simulink model "P170_PV_MPPT_Integration"  (R2026b)
settings: Solver=FixedStepDiscrete  StopTime=2  FixedStep=P170_dt
values from neighbouring files (symbols this model uses):
  P170_Imp = im(ix)    [P170_PV_Initialize.m]
  P170_Vmp = vm(ix)    [P170_PV_Initialize.m]
undefined symbols (not defined in the file or in its folder): P170_T
libraries: fl_lib x4, nesl_utility x2, ee_lib x1
settings Model: Creator=simay  LastModifiedBy=aj26g
settings SimscapeCC: SimscapeLogType=all  SimscapeNominalValues="[{\"value\":\"1\",\"unit\":\"A\"},{\"value\":\"1\",\"unit\":\"bar\"},{\"value\":\"1\",\"unit\":\"cm^2\"},{\"value\":\"1\",\"unit\":\"cm^3/s\"},{\"value\":\"1\",\"unit\":\"kJ/kg\"},{\"value\":\"1\",\"unit\":\"kW\"},{\"value\":\"1\",\"unit\":\"l\"},{\"value\":\"1\",\"unit\":\"N\"},{\"value\":\"1\",\"unit\":\"N*m\"},{\"value\":\"1\",\"unit\":\"V\"},{\"value\":\"0.001\",\"unit\":\"Wb\"}]"  SimscapeUseEnergyAccounting=off

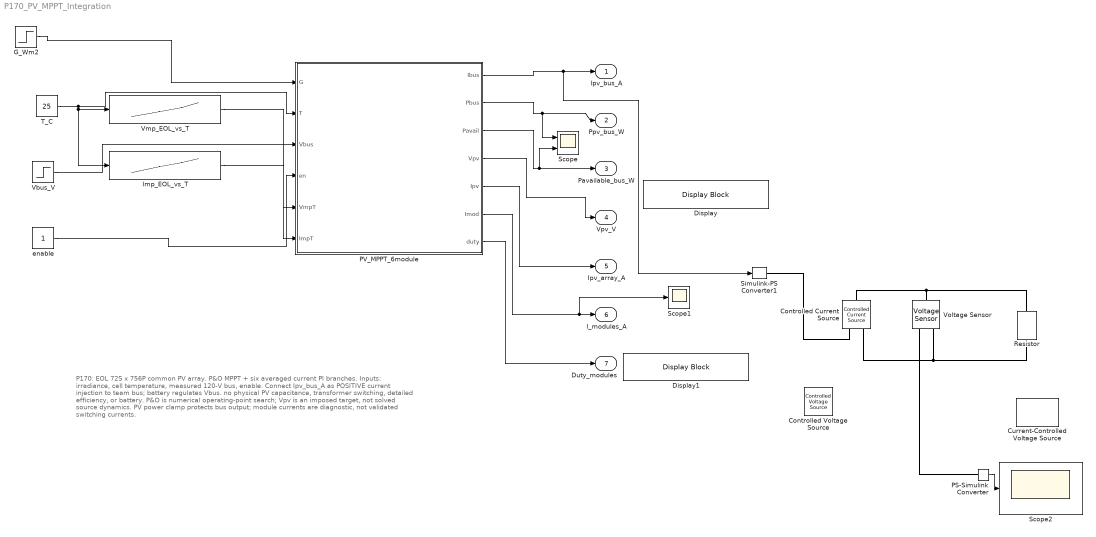
== system P170_PV_MPPT_Integration ==
  note: P170: EOL 72S x 756P common PV array. P&O MPPT + six averaged current PI branches.
      | Inputs: irradiance, cell temperature, measured 120-V bus, enable.
      | Connect Ipv_bus_A as POSITIVE current injection to team bus; battery regulates Vbus.
      |
      | no physical PV capacitance, transformer switching, detailed efficiency, or battery.
      | P&O is numerical operating-point search; Vpv is an imposed target, not solved source dynamics.
      | PV power clamp protects bus output; module currents are diagnostic, not validated switching currents.
  Controlled Current Source : fl_lib/Electrical/Electrical Sources/Controlled Current Source
  Controlled Voltage Source : fl_lib/Electrical/Electrical Sources/Controlled Voltage Source
  Current-Controlled Voltage Source : fl_lib/Electrical/Electrical Sources/Current-Controlled Voltage Source  K=1 Ohm  i1_specify=off  i1_priority=None  i1=0 A  i1_nominal_specify=off  i1_nominal_value=1  i1_nominal_unit=A  v2_specify=off  v2_priority=None  v2=0 V  v2_nominal_specify=off  v2_nominal_value=1  v2_nominal_unit=V
  Display : DisplayBlock  LabelPosition=Hide  Transparency=1  GridColor=[0.502, 0.502, 0.502]
  Display1 : DisplayBlock  LabelPosition=Hide  Transparency=1  GridColor=[0.502, 0.502, 0.502]
  G_Wm2 : Step  Time=0.8  InitialValue=1367  FinalValue=700  SampleTime=0
  Imp_EOL_vs_T : Lookup_n-D  NumberOfTableDimensions=1  BreakpointsForDimension1=P170_T  Table=P170_Imp  InternalRulePriority=Speed  RndMeth=Simplest
  PS-Simulink Converter : nesl_utility/PS-Simulink Converter  PhysicalDomain=network_engine_domain  SubClassName=ps_output  LeftPortType=input  RightPortType=output  PseudoPeriodic=off  Frequencies=[]  VectorFormat=inherit  Unit=inherit  AffineConversion=off
  PV_MPPT_6module : MATLAB Function  TreatAsAtomicUnit=on
  Resistor : ee_lib/Passive/Resistor  R=30000 Ohm  enable_R_tol=ee.enum.toleranceApplication.none  R_tol=5  tol_distribution=ee.enum.toleranceDistribution.uniform  nSigma=4  enable_operating_limits=ee.enum.enable.no  operating_limit_action=ee.enum.passive.reportOpLim.warn  power_rating=1 W  max_working_voltage=100 V  noise_mode=ee.enum.sources.noise.Disabled  Tdevice=25 degC  sample_time=1e-3 s  repeatability=ee.enum.ic.repeatability.notRepeatable  user_seed=0  auto_seed=4111000739  power_derating_T1=70 degC  power_derating_T2=155 degC  operating_temperature_range_vec=[-50, 150] degC  alpha=3.93e-3 1/K  Tmeas=25 degC  thermal_mass=100 J/K  temperature_specify=off  temperature_priority=High  temperature=298.15 K  temperature_nominal_specify=off  temperature_nominal_value=1  temperature_nominal_unit=K
  Scope : Scope  NumInputPorts=2
      settings: ActiveDisplayYMinimum=-1.4996053799360058  ActiveDisplayYMaximum=1.4239551585454688
  Scope1 : Scope
      settings: ActiveDisplayYMinimum=25.569170414602688  ActiveDisplayYMaximum=92.411823172385326
  Scope2 : Scope
      settings: DataLoggingVariableName=ScopeData2
  Simulink-PS Converter1 : nesl_utility/Simulink-PS Converter  PhysicalDomain=network_engine_domain  SubClassName=ps_input  LeftPortType=input  RightPortType=output  PseudoPeriodic=off  Frequencies=[]  NoiseDistribution=none  NoiseParameters=[]  Unit=1  AffineConversion=off  FilteringAndDerivatives=provide  SimscapeFilterOrder=1  InputFilterTimeConstant=0.001  UdotUserProvided=0
  T_C : Constant  Value=25
  Vbus_V : Step  Time=1.2  InitialValue=120  FinalValue=115  SampleTime=0
  Vmp_EOL_vs_T : Lookup_n-D  NumberOfTableDimensions=1  BreakpointsForDimension1=P170_T  Table=P170_Vmp  InternalRulePriority=Speed  RndMeth=Simplest
  Voltage Sensor : fl_lib/Electrical/Electrical Sensors/Voltage Sensor
  enable : Constant
  Ipv_bus_A : Outport
  Ppv_bus_W : Outport  Port=2
  Pavailable_bus_W : Outport  Port=3
  Vpv_V : Outport  Port=4
  Ipv_array_A : Outport  Port=5
  I_modules_A : Outport  Port=6
  Duty_modules : Outport  Port=7
  wires:
  G_Wm2/1 -> PV_MPPT_6module/1(G)
  T_C/1 -> Vmp_EOL_vs_T/1, Imp_EOL_vs_T/1, PV_MPPT_6module/2(T)
  Vbus_V/1 -> PV_MPPT_6module/3(Vbus)
  enable/1 -> PV_MPPT_6module/4(en)
  Vmp_EOL_vs_T/1 -> PV_MPPT_6module/5(VmpT)
  Imp_EOL_vs_T/1 -> PV_MPPT_6module/6(ImpT)
  PV_MPPT_6module/1(Ibus) -> Simulink-PS Converter1/1, Ipv_bus_A/1
  PV_MPPT_6module/3(Pavail) -> Scope/2, Pavailable_bus_W/1
  PV_MPPT_6module/4(Vpv) -> Vpv_V/1
  PV_MPPT_6module/5(Ipv) -> Ipv_array_A/1
  PV_MPPT_6module/6(Imod) -> Scope1/1, I_modules_A/1
  PV_MPPT_6module/7(duty) -> Duty_modules/1
  PV_MPPT_6module/2(Pbus) -> Scope/1, Ppv_bus_W/1
  PS-Simulink Converter/1 -> Scope2/1
  connections:
  Controlled Current Source/RConn1 -- Simulink-PS Converter1/RConn1
  Resistor/LConn1 -- Controlled Current Source/LConn1 -- Voltage Sensor/LConn1
  Controlled Current Source/RConn2 -- Voltage Sensor/RConn2 -- Resistor/RConn1
  PS-Simulink Converter/LConn1 -- Voltage Sensor/RConn1

== matlab function P170_PV_MPPT_Integration/PV_MPPT_6module ==
  data: G input; Ibus output; T input; Vbus input; en input; VmpT input; ImpT input; Pbus output; Pavail output; Vpv output; Ipv output; Imod output; duty output
function [Ibus, Pbus, Pavail, Vpv, Ipv, Imod, duty] = fcn(G,T,Vbus,en,VmpT,ImpT)
%#codegen
% EOL teammate MPP data; illustrative piecewise I-V fit.
% Shared PV bus, single coordinated P&O, six averaged PI branches.
persistent Vcmd dir Pprev count il integ
if isempty(Vcmd)
 Vcmd=217; dir=1; Pprev=0; count=0; il=zeros(6,1); integ=zeros(6,1);
end
dt=1e-4; eta=0.96; Gref=1367;
gs=max(0,min(1.5,G/Gref));
vmp=max(10,VmpT); imp=max(0,ImpT)*gs;
% Curve passes through Isc, Imp at Vmp, and zero at Voc.
% Isc=1.04 Imp, Voc=1.13 Vmp are MODEL ASSUMPTIONS.
isc=1.04*imp; voc=1.13*vmp;
Vcmd=max(0.5*vmp,min(0.99*voc,Vcmd));
if Vcmd<=vmp
 ipv=max(0,isc-(isc-imp)*(Vcmd/vmp)^2);
else
 ipv=max(0,imp*(voc-Vcmd)/(voc-vmp));
end
Ppv=Vcmd*ipv; Pavail=max(0,vmp*imp*eta);
count=count+1;
if count>=100
 if Ppv<Pprev, dir=-dir; end
 Vcmd=Vcmd+dir*0.5; Pprev=Ppv; count=0;
end
% Power-to-current reference; current limited by PV production.
v=max(30,Vbus);
Ptarget=max(0,min(Ppv*eta,Pavail))*max(0,min(1,en));
Iref=Ptarget/v/6;
Imod=zeros(6,1); duty=zeros(6,1);
for k=1:6
 % Averaged current PI with feedforward; shared-array duty proxy.
 err=Iref-il(k);
 dff=Vbus/max(1,1.15*Vcmd);
 d=max(0,min(0.85,dff+0.0015*err+integ(k)));
 % Average inductor dynamics; 33 uH each.
 next=il(k)+dt*(1.15*Vcmd*d-Vbus)/33e-6;
 % Avoid nonphysical reverse PV current.
 next=max(0,next);
 % Anti-windup: integrate only when unsaturated or correcting.
 if (d>0 && d<0.85) || (d<=0 && err>0) || (d>=0.85 && err<0)
  integ(k)=integ(k)+3*dt*err;
 end
 il(k)=next; Imod(k)=next; duty(k)=d;
end
% Conservation clamp: do not inject more power than PV can supply.
Iraw=sum(Imod); Ibus=min(Iraw,Ptarget/v);
Pbus=Ibus*max(0,Vbus); Vpv=Vcmd; Ipv=ipv;
end
